simulink model "single_phase_afe"  (R2026b)
settings: Solver=ode23tb  StopTime=param.sim.simlength  FixedStep=param.sim.tc  MaxStep=param.glb_time.tc
values from neighbouring files (symbols this model uses):
  param = struct()    [init_model.m]
undefined symbols (not defined in the file or in its folder): magnitude
libraries: fl_lib x201, nesl_utility x108, igbt_simple_2th_lib x8, single_phase_pwm_modulator x2, dq_vector_pi x2, phase_shift_filter_ccaller x2, pi_ctrl x2, discrete_time_low_pass_filter x2, lithium_ion_battery x1, dclink_for_two_levels x1, three_phase_voltage_with_frt_emulator x1, simulink x1
(part 2 of 7)

== system single_phase_afe/grid/grid_emulator/threephase_vi_measures ==
  Bus Creator : BusCreator  Inputs=6
  Current Sensor : fl_lib/Electrical/Electrical Sensors/Current Sensor
  Current Sensor1 : fl_lib/Electrical/Electrical Sensors/Current Sensor
  Current Sensor2 : fl_lib/Electrical/Electrical Sensors/Current Sensor
  Electrical Reference1 : fl_lib/Electrical/Electrical Elements/Electrical Reference
  Voltage Sensor : fl_lib/Electrical/Electrical Sensors/Voltage Sensor
  Voltage Sensor1 : fl_lib/Electrical/Electrical Sensors/Voltage Sensor
  Voltage Sensor2 : fl_lib/Electrical/Electrical Sensors/Voltage Sensor
  i : Selector  InputPortWidth=6  IndexOptions=Index vector (dialog)  Indices=[4 5 6]  OutputSizes=1  RuntimeRangeChecks=off
  ia_grid : nesl_utility/PS-Simulink Converter  PhysicalDomain=network_engine_domain  SubClassName=ps_output  LeftPortType=input  RightPortType=output  PseudoPeriodic=off  Frequencies=[]  VectorFormat=1-D array  Unit=A  AffineConversion=off
  ib_grid : nesl_utility/PS-Simulink Converter  PhysicalDomain=network_engine_domain  SubClassName=ps_output  LeftPortType=input  RightPortType=output  PseudoPeriodic=off  Frequencies=[]  VectorFormat=1-D array  Unit=A  AffineConversion=off
  ic_grid : nesl_utility/PS-Simulink Converter  PhysicalDomain=network_engine_domain  SubClassName=ps_output  LeftPortType=input  RightPortType=output  PseudoPeriodic=off  Frequencies=[]  VectorFormat=1-D array  Unit=A  AffineConversion=off
  u : Selector  InputPortWidth=6  IndexOptions=Index vector (dialog)  Indices=[1 2 3]  OutputSizes=1  RuntimeRangeChecks=off
  ua_grid : nesl_utility/PS-Simulink Converter  PhysicalDomain=network_engine_domain  SubClassName=ps_output  LeftPortType=input  RightPortType=output  PseudoPeriodic=off  Frequencies=[]  VectorFormat=1-D array  Unit=V  AffineConversion=off
  ub_grid : nesl_utility/PS-Simulink Converter  PhysicalDomain=network_engine_domain  SubClassName=ps_output  LeftPortType=input  RightPortType=output  PseudoPeriodic=off  Frequencies=[]  VectorFormat=1-D array  Unit=V  AffineConversion=off
  uc_grid : nesl_utility/PS-Simulink Converter  PhysicalDomain=network_engine_domain  SubClassName=ps_output  LeftPortType=input  RightPortType=output  PseudoPeriodic=off  Frequencies=[]  VectorFormat=1-D array  Unit=V  AffineConversion=off
  Ua : PMIOPort  Side=Left
  ua : PMIOPort  Port=2  Side=Right
  Ub : PMIOPort  Port=3  Side=Left
  ub : PMIOPort  Port=4  Side=Right
  Uc : PMIOPort  Port=5  Side=Left
  uc : PMIOPort  Port=6  Side=Right
  tag scope: i_abc_line=global, u_abc_line=global
  wires:
  Bus Creator/1 -> i/1, u/1  "vi_data"
  ib_grid/1 -> Bus Creator/5  "ib"
  ia_grid/1 -> Bus Creator/4  "ia"
  ic_grid/1 -> Bus Creator/6  "ic"
  ua_grid/1 -> Bus Creator/1  "ua"
  ub_grid/1 -> Bus Creator/2  "ub"
  uc_grid/1 -> Bus Creator/3  "uc"
  i/1 -> [i_abc_line]
  u/1 -> [u_abc_line]
  connections:
  Current Sensor1/LConn1 -- Ub/RConn1 -- Voltage Sensor1/LConn1
  Electrical Reference1/LConn1 -- Voltage Sensor/RConn2 -- Voltage Sensor2/RConn2 -- Voltage Sensor1/RConn2
  Voltage Sensor/RConn1 -- ua_grid/LConn1
  Current Sensor/RConn2 -- ua/RConn1
  Voltage Sensor1/RConn1 -- ub_grid/LConn1
  Voltage Sensor2/LConn1 -- Current Sensor2/LConn1 -- Uc/RConn1
  Current Sensor/LConn1 -- Ua/RConn1 -- Voltage Sensor/LConn1
  Current Sensor1/RConn2 -- ub/RConn1
  Voltage Sensor2/RConn1 -- uc_grid/LConn1
  ib_grid/LConn1 -- Current Sensor1/RConn1
  ia_grid/LConn1 -- Current Sensor/RConn1
  ic_grid/LConn1 -- Current Sensor2/RConn1
  Current Sensor2/RConn2 -- uc/RConn1

== system single_phase_afe/single_phase_inverter/single phase inverter control/acquisition_and_scaling_current_buffer ==
  in : Inport
  1/Ti5 : Gain  Gain=1/param.afe.buffer.ibez  SaturateOnIntegerOverflow=on  OutDataTypeStr=Inherit: Same as input  ParamDataTypeStr=Inherit: Same as input
  Quantizer : Quantizer  QuantizationInterval=param.meas.adc_quantization
  out : Outport
  wires:
  in/1 -> 1/Ti5/1
  1/Ti5/1 -> Quantizer/1
  Quantizer/1 -> out/1

== system single_phase_afe/single_phase_inverter/single phase inverter control/acquisition_and_scaling_current_with_white_noise ==
  in : Inport
  1/Ti5 : Gain  Gain=1/param.afe.hw.ibez  SaturateOnIntegerOverflow=on  OutDataTypeStr=Inherit: Same as input  ParamDataTypeStr=Inherit: Same as input
  Band-Limited White Noise : simulink/Sources/Band-Limited White Noise  Commented=on  Cov=1e-10  Ts=param.glb_time.tc  seed=[23341]
  Quantizer : Quantizer  QuantizationInterval=param.meas.adc_quantization
  Sum : Sum  Inputs=|++
  current_measure_with-without noise : Scope  NumInputPorts=2
      settings: ActiveDisplayYMinimum=-1.259685411609524  ActiveDisplayYMaximum=1.2603394332468927  DataLoggingVariableName=ScopeData15
  out : Outport
  wires:
  in/1 -> 1/Ti5/1
  1/Ti5/1 -> Sum/1, current_measure_with-without noise/1  "iload_without_noise"
  Sum/1 -> Quantizer/1
  Band-Limited White Noise/1 -> Sum/2
  Quantizer/1 -> out/1, current_measure_with-without noise/2  "iload_with_noise"

== system single_phase_afe/single_phase_inverter/single phase inverter control/acquisition_and_scaling_dc_voltage ==
  in : Inport
  1/Ti3 : Gain  Gain=1/param.afe.hw.udc_nom  SaturateOnIntegerOverflow=on  OutDataTypeStr=Inherit: Same as input  ParamDataTypeStr=Inherit: Same as input
  Quantizer : Quantizer  QuantizationInterval=param.meas.adc_quantization
  out : Outport
  wires:
  in/1 -> 1/Ti3/1
  1/Ti3/1 -> Quantizer/1
  Quantizer/1 -> out/1

== system single_phase_afe/single_phase_inverter/single phase inverter control/acquisition_and_scaling_dc_voltage_buffer ==
  in : Inport
  1/Ti3 : Gain  Gain=1/param.afe.hw.udc_nom  SaturateOnIntegerOverflow=on  OutDataTypeStr=Inherit: Same as input  ParamDataTypeStr=Inherit: Same as input
  Quantizer : Quantizer  QuantizationInterval=param.meas.adc_quantization
  out : Outport
  wires:
  Quantizer/1 -> out/1
  1/Ti3/1 -> Quantizer/1
  in/1 -> 1/Ti3/1

== system single_phase_afe/single_phase_inverter/single phase inverter control/acquisition_and_scaling_grid_voltage_ac ==
  in : Inport
  1/Ti5 : Gain  Gain=1/param.grid.emu.u2bez  SaturateOnIntegerOverflow=on  OutDataTypeStr=Inherit: Same as input  ParamDataTypeStr=Inherit: Same as input
  Quantizer : Quantizer  QuantizationInterval=param.meas.adc_quantization
  out : Outport
  wires:
  Quantizer/1 -> out/1
  1/Ti5/1 -> Quantizer/1
  in/1 -> 1/Ti5/1

== system single_phase_afe/single_phase_inverter/single phase inverter control/acquisition_and_scaling_voltage ==
  in : Inport
  1/Ti5 : Gain  Gain=1/param.afe.hw.ubez  SaturateOnIntegerOverflow=on  OutDataTypeStr=Inherit: Same as input  ParamDataTypeStr=Inherit: Same as input
  Quantizer : Quantizer  QuantizationInterval=param.meas.adc_quantization
  pwm filtering for measure : cstblocks_lti/LTI System  sys=param.afe.ctrl.sogi.flt_beta  IC=[]  PadeOrder=0
  out : Outport
  wires:
  in/1 -> 1/Ti5/1
  pwm filtering for measure/1 -> Quantizer/1
  1/Ti5/1 -> pwm filtering for measure/1
  Quantizer/1 -> out/1

== system single_phase_afe/single_phase_inverter/single phase inverter control/pwm modulator ==
  vout : Inport
  Constant : Constant  Value=0
  Single phase two level PWM generator with global TRGO : single_phase_pwm_modulator/Single phase two level PWM generator with global TRGO  f=param.glb_time.fPWM_AFE  m_up=0.98  m_low=0.02  dead_time=param.glb_time.dead_time_AFE  pos_cmd_gate=18  neg_cmd_gate=-3  polarity=-1  tc=param.glb_time.tc  double_sampling=param.glb_time.TRGO_AFE_double_update
  gate_cmds : Outport
  tag scope: TRGO_AFE_1=global
  wires:
  vout/1 -> Single phase two level PWM generator with global TRGO/3
  Constant/1 -> Single phase two level PWM generator with global TRGO/2
  Single phase two level PWM generator with global TRGO/2 -> gate_cmds/1
  Single phase two level PWM generator with global TRGO/1 -> [TRGO_AFE_1]
  [time_afe_module_1] -> Single phase two level PWM generator with global TRGO/1

== system single_phase_afe/single_phase_inverter/single phase inverter control/pwm modulator_dclink_compensator ==
  vout : Inport
  Constant : Constant  Value=0
  Single phase two level PWM generator with global TRGO : single_phase_pwm_modulator/Single phase two level PWM generator with global TRGO  f=param.glb_time.fPWM_AFE  m_up=0.98  m_low=0.02  dead_time=param.glb_time.dead_time_AFE  pos_cmd_gate=18  neg_cmd_gate=-3  polarity=-1  tc=param.glb_time.tc  double_sampling=param.glb_time.TRGO_AFE_double_update
  gate_cmds : Outport
  wires:
  [time_afe_module_1] -> Single phase two level PWM generator with global TRGO/1
  Single phase two level PWM generator with global TRGO/2 -> gate_cmds/1
  Constant/1 -> Single phase two level PWM generator with global TRGO/2
  vout/1 -> Single phase two level PWM generator with global TRGO/3

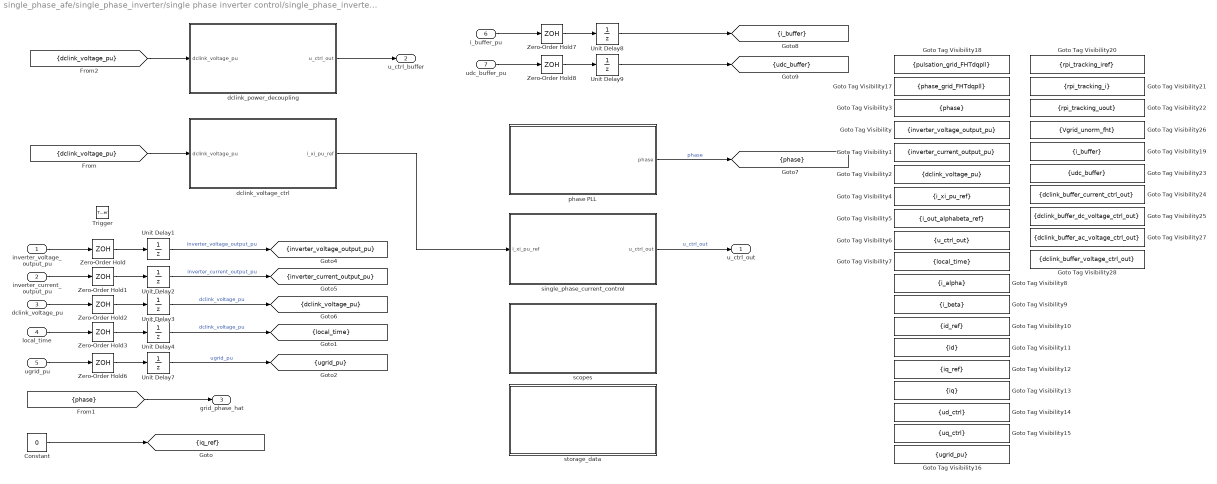
== system single_phase_afe/single_phase_inverter/single phase inverter control/single_phase_inverter_ctrl ==
  inverter_voltage_output_pu : Inport
  inverter_current_output_pu : Inport  Port=2
  dclink_voltage_pu : Inport  Port=3
  local_time : Inport  Port=4
  ugrid_pu : Inport  Port=5
  i_buffer_pu : Inport  Port=6
  udc_buffer_pu : Inport  Port=7
  Trigger : TriggerPort  VariantControl=(inherit)  PortDimensions=1
  Constant : Constant  Value=0
  Goto Tag Visibility : GotoTagVisibility  GotoTag=inverter_voltage_output_pu
  Goto Tag Visibility1 : GotoTagVisibility  GotoTag=inverter_current_output_pu
  Goto Tag Visibility10 : GotoTagVisibility  GotoTag=id_ref
  Goto Tag Visibility11 : GotoTagVisibility  GotoTag=id
  Goto Tag Visibility12 : GotoTagVisibility  GotoTag=iq_ref
  Goto Tag Visibility13 : GotoTagVisibility  GotoTag=iq
  Goto Tag Visibility14 : GotoTagVisibility  GotoTag=ud_ctrl
  Goto Tag Visibility15 : GotoTagVisibility  GotoTag=uq_ctrl
  Goto Tag Visibility16 : GotoTagVisibility  GotoTag=ugrid_pu
  Goto Tag Visibility17 : GotoTagVisibility  GotoTag=phase_grid_FHTdqpll
  Goto Tag Visibility18 : GotoTagVisibility  GotoTag=pulsation_grid_FHTdqpll
  Goto Tag Visibility19 : GotoTagVisibility  GotoTag=i_buffer
  Goto Tag Visibility2 : GotoTagVisibility  GotoTag=dclink_voltage_pu
  Goto Tag Visibility20 : GotoTagVisibility  GotoTag=rpi_tracking_iref
  Goto Tag Visibility21 : GotoTagVisibility  GotoTag=rpi_tracking_i
  Goto Tag Visibility22 : GotoTagVisibility  GotoTag=rpi_tracking_uout
  Goto Tag Visibility23 : GotoTagVisibility  GotoTag=udc_buffer
  Goto Tag Visibility24 : GotoTagVisibility  GotoTag=dclink_buffer_current_ctrl_out
  Goto Tag Visibility25 : GotoTagVisibility  GotoTag=dclink_buffer_dc_voltage_ctrl_out
  Goto Tag Visibility26 : GotoTagVisibility  GotoTag=Vgrid_unorm_fht
  Goto Tag Visibility27 : GotoTagVisibility  GotoTag=dclink_buffer_ac_voltage_ctrl_out
  Goto Tag Visibility28 : GotoTagVisibility  GotoTag=dclink_buffer_voltage_ctrl_out
  Goto Tag Visibility3 : GotoTagVisibility  GotoTag=phase
  Goto Tag Visibility4 : GotoTagVisibility  GotoTag=i_xi_pu_ref
  Goto Tag Visibility5 : GotoTagVisibility  GotoTag=i_out_alphabeta_ref
  Goto Tag Visibility6 : GotoTagVisibility  GotoTag=u_ctrl_out
  Goto Tag Visibility7 : GotoTagVisibility  GotoTag=local_time
  Goto Tag Visibility8 : GotoTagVisibility  GotoTag=i_alpha
  Goto Tag Visibility9 : GotoTagVisibility  GotoTag=i_beta
  Unit Delay{1..4,7..9} (7 alike) : UnitDelay  SampleTime=-1
  Zero-Order Hold{,1..3,6..8} (7 alike) : ZeroOrderHold  SampleTime=-1
  dclink_power_decoupling : Subsystem
  dclink_voltage_ctrl : Subsystem
  phase PLL : Subsystem
  scopes : Subsystem
  single_phase_current_control : Subsystem
  storage_data : Subsystem
  u_ctrl_out : Outport
  u_ctrl_buffer : Outport  Port=2
  grid_phase_hat : Outport  Port=3
  tag scope: dclink_voltage_pu=scoped, i_buffer=scoped, inverter_current_output_pu=scoped, inverter_voltage_output_pu=scoped, iq_ref=scoped, local_time=scoped, phase=scoped, udc_buffer=scoped, ugrid_pu=scoped
  wires:
  inverter_voltage_output_pu/1 -> Zero-Order Hold/1
  inverter_current_output_pu/1 -> Zero-Order Hold1/1
  dclink_voltage_pu/1 -> Zero-Order Hold2/1
  Unit Delay1/1 -> [inverter_voltage_output_pu]  "inverter_voltage_output_pu"
  Unit Delay2/1 -> [inverter_current_output_pu]  "inverter_current_output_pu"
  Unit Delay3/1 -> [dclink_voltage_pu]  "dclink_voltage_pu"
  phase PLL/1(phase) -> [phase]  "phase"
  single_phase_current_control/1(u_ctrl_out) -> u_ctrl_out/1  "u_ctrl_out"
  Zero-Order Hold/1 -> Unit Delay1/1
  Zero-Order Hold1/1 -> Unit Delay2/1
  Zero-Order Hold2/1 -> Unit Delay3/1
  Zero-Order Hold3/1 -> Unit Delay4/1
  Unit Delay4/1 -> [local_time]  "dclink_voltage_pu"
  local_time/1 -> Zero-Order Hold3/1
  ugrid_pu/1 -> Zero-Order Hold6/1
  Zero-Order Hold6/1 -> Unit Delay7/1
  Unit Delay7/1 -> [ugrid_pu]  "ugrid_pu"
  [dclink_voltage_pu] -> dclink_voltage_ctrl/1(dclink_voltage_pu)
  dclink_voltage_ctrl/1(i_xi_pu_ref) -> single_phase_current_control/1(i_xi_pu_ref)
  [phase] -> grid_phase_hat/1
  [dclink_voltage_pu] -> dclink_power_decoupling/1(dclink_voltage_pu)
  dclink_power_decoupling/1(u_ctrl_out) -> u_ctrl_buffer/1
  Zero-Order Hold7/1 -> Unit Delay8/1
  i_buffer_pu/1 -> Zero-Order Hold7/1
  Unit Delay8/1 -> [i_buffer]
  Unit Delay9/1 -> [udc_buffer]
  udc_buffer_pu/1 -> Zero-Order Hold8/1
  Zero-Order Hold8/1 -> Unit Delay9/1
  Constant/1 -> [iq_ref]

== system single_phase_afe/single_phase_inverter/single_phase_inverter/single phase inverter ==
  gate_cmds : Inport
  three_phase_inverter_with_igbt_simple_2th : Subsystem
  uac_out(+) : PMIOPort  Side=Left
  uac_out(-) : PMIOPort  Port=2  Side=Left
  udc(+) : PMIOPort  Port=3  Side=Right
  udc(-) : PMIOPort  Port=4  Side=Right
  wires:
  gate_cmds/1 -> three_phase_inverter_with_igbt_simple_2th/1(gate_cmds)
  connections:
  udc(-)/RConn1 -- three_phase_inverter_with_igbt_simple_2th/LConn2
  udc(+)/RConn1 -- three_phase_inverter_with_igbt_simple_2th/LConn1
  uac_out(+)/RConn1 -- three_phase_inverter_with_igbt_simple_2th/RConn1
  uac_out(-)/RConn1 -- three_phase_inverter_with_igbt_simple_2th/RConn2

== system single_phase_afe/dclink_buffer_ctrl/single_phase_inverter/single phase inverter/three_phase_inverter_with_igbt_simple_2th ==
  gate_cmds : Inport
  full_bridge_with_igbt_simple_2th : Subsystem  mask{vce_sat_m=param.afe.igbt.Vce_sat, v_gamma_m=param.afe.igbt.Vdon_diode, Vth_gate_m=param.afe.igbt.Vth, Vth_gate_hyst_m=0.85, Eon_m=param.afe.igbt.Eon*1000, Eoff_m=param.afe.igbt.Eoff*1000, Err_m=param.afe.igbt.Erec*1000, Ic_ref_m=param.afe.igbt.Ion_sw_losses, Vdc_ref_m=param.afe.igbt.Voff_sw_losses, Vblock_Errf_m=50, rce_on_m=param.afe.igbt.Rce_on*1000, rd_on_m=param.afe.igbt.Rdon_diode*1000, Gce_off_m=1e-6, time_constant_edge_m=param.glb_time.tc, time_constant_ploss_m=1e3, Csnubber_m=param.afe.igbt.Csnubber_zvs, Rsnubber_m=param.afe.igbt.Rsnubber_zvs, rth_switch_JH_m=param.afe.igbt.Rth_switch_JH, rth_switch_HA_m=param.thermal.heatsink.Rth_switch_HA, rth_diode_JH_m=param.afe.igbt.Rth_diode_JH, rth_diode_HA_m=param.thermal.heatsink.Rth_diode_HA, JunctionTermalMass_m=param.afe.igbt.JunctionTermalMass, Tambient_m=param.thermal.Tambient, mass_heatsink_m=param.thermal.heatsink.no_weight, specific_heat_m=param.thermal.heatsink.cp}
      mask prompts: vce_sat_m "Collector-emitter on-stage voltage [V]"; v_gamma_m "Diode forward voltage [V]"; Vth_gate_m "Gate-emitter threshold voltage [V]"; Vth_gate_hyst_m "Half hysteresis band for the switching events [V]"; Eon_m "Turn-on energy at Ic_ref, Vdc_ref [mJ]"; Eoff_m "Turn-off energy at Ic_ref, Vdc_ref [mJ]"; Err_m "Reverse recovery energy at Ic_ref, Vdc_ref [mJ]"; Ic_ref_m "Reference current of the energies [A]"; Vdc_ref_m "Reference voltage of the energies [V]"; Vblock_Errf_m "V block Err"; rce_on_m "IGBT on-state series resistance [mOhm]"; rd_on_m "Diode series resistance [mOhm]"; Gce_off_m "Off-state conductance [1/Ohm]"; time_constant_edge_m "Sample&hold time constant (<< on-time) [us]"; time_constant_ploss_m "Loss averaging time constant (2-5 x Tsw) [us]"; Csnubber_m "Csnubber [F]"; Rsnubber_m "Rsnubber [Ohm]"; rth_switch_JH_m "Thermal impedance Junction-heatsink switch [K/W]"; rth_switch_HA_m "Thermal impedance heatsink-ambient switch[K/W]"; rth_diode_JH_m "Thermal impedance Junction-heatsink diode [K/W]"; rth_diode_HA_m "Thermal impedance heatsink-ambient diode [K/W]"; JunctionTermalMass_m "Junction Thermal Mass [J/K]"; Tambient_m "Ambient temperature [degC]"; mass_heatsink_m "Mass heatsink [kg]"; specific_heat_m "Specific heat capacity of the heatsink [J/K/Kg]"
  u1 : PMIOPort  Side=Right
  u2 : PMIOPort  Port=2  Side=Right
  udc(+) : PMIOPort  Port=3  Side=Left
  udc(-) : PMIOPort  Port=4  Side=Left
  wires:
  gate_cmds/1 -> full_bridge_with_igbt_simple_2th/1(gate_cmds)
  connections:
  u1/RConn1 -- full_bridge_with_igbt_simple_2th/RConn1
  u2/RConn1 -- full_bridge_with_igbt_simple_2th/RConn2
  udc(-)/RConn1 -- full_bridge_with_igbt_simple_2th/LConn2
  udc(+)/RConn1 -- full_bridge_with_igbt_simple_2th/LConn1

== system single_phase_afe/single_phase_inverter/single phase inverter control/single_phase_inverter_ctrl/dclink_power_decoupling ==
  dclink_voltage_pu : Inport
  dclink_decoupling_ctrl : Subsystem
  idc_buffer_ctrl : Subsystem
  udc_buffer_ctrl : Subsystem
  u_ctrl_out : Outport
  wires:
  idc_buffer_ctrl/1(u_ctrl_out) -> u_ctrl_out/1, dclink_decoupling_ctrl/3(u_ctrl_out)  "u_ctrl_out"
  [udc_buffer] -> udc_buffer_ctrl/1(udc_buffer_pu)
  udc_buffer_ctrl/1(i_dc_buffer_ref) -> dclink_decoupling_ctrl/1(i_dc_buffer_ref)  "i_dc_buffer_ref"
  dclink_voltage_pu/1 -> dclink_decoupling_ctrl/2(udc_dclink_pu)  "udc_dclink_pu"
  dclink_decoupling_ctrl/1(i_buffer_ref) -> idc_buffer_ctrl/1(i_buffer_ref)  "i_buffer_ref"

== system single_phase_afe/single_phase_inverter/single phase inverter control/single_phase_inverter_ctrl/dclink_voltage_ctrl ==
  dclink_voltage_pu : Inport
  1/Ti : Gain  Gain=param.afe.ctrl.kp_udc  SaturateOnIntegerOverflow=on  OutDataTypeStr=Inherit: Same as input  ParamDataTypeStr=Inherit: Same as input
  Gain : Gain  Gain=-1
  Saturation : Saturate  UpperLimit=param.afe.ctrl.i_ref_lim  LowerLimit=-param.afe.ctrl.i_ref_lim
  Sum1 : Sum  Inputs=+++  SaturateOnIntegerOverflow=on
  Sum2 : Sum  Inputs=-+  SaturateOnIntegerOverflow=on
  Sum3 : Sum  Inputs=-+  SaturateOnIntegerOverflow=on
  To Workspace1 : ToWorkspace  VariableName=udc_pu_sim_mod1  SampleTime=-1
      settings: MaxDataPoints=param.glb_time.Ns_afe
  To Workspace3 : ToWorkspace  VariableName=udc_pu_ref_sim_mod1  SampleTime=-1
      settings: MaxDataPoints=param.glb_time.Ns_afe
  Unit Delay4 : UnitDelay  SampleTime=-1
  discrete-time-low-pass-filter1 : discrete_time_low_pass_filter/discrete-time-low-pass-filter  tau=param.afe.ctrl.tau_udc_ref  ts=param.glb_time.ts_afe
  kp : Gain  Gain=param.afe.ctrl.ki_udc*param.glb_time.ts_afe  SaturateOnIntegerOverflow=on  OutDataTypeStr=Inherit: Same as input  ParamDataTypeStr=Inherit: Same as input
  udc_norm_ref : Step  Time=param.afe.ctrl.t_udc_ref  FinalValue=param.afe.ctrl.udc_pu_ref
  udc_tracking : Scope  NumInputPorts=3
      settings: ActiveDisplayYMinimum=-2.0073730468749997  ActiveDisplayYMaximum=1.5663574218749998  DataLoggingVariableName=ScopeData8
  i_xi_pu_ref : Outport
  wires:
  1/Ti/1 -> Sum1/1, Sum3/1
  kp/1 -> Sum1/2
  Sum3/1 -> Unit Delay4/1
  Unit Delay4/1 -> Sum1/3
  udc_norm_ref/1 -> discrete-time-low-pass-filter1/1
  dclink_voltage_pu/1 -> Sum2/1, To Workspace1/1, udc_tracking/2  "udc_pu"
  Sum2/1 -> kp/1, 1/Ti/1
  Sum1/1 -> Saturation/1
  Saturation/1 -> Sum3/2, Gain/1
  Gain/1 -> udc_tracking/3, i_xi_pu_ref/1  "i_xi_pu_ref"
  discrete-time-low-pass-filter1/1 -> To Workspace3/1, udc_tracking/1, Sum2/2  "udc_pu_ref"

== system single_phase_afe/single_phase_inverter/single phase inverter control/single_phase_inverter_ctrl/phase PLL ==
  FHT-PLL : Subsystem
  FHTdqpll : Scope  NumInputPorts=2
      settings: ActiveDisplayYMinimum=-1.624956414103508  ActiveDisplayYMaximum=4.624995157122612  DataLoggingVariableName=ScopeData3
  phase : Outport
  tag scope: phase_grid_FHTdqpll=scoped, pulsation_grid_FHTdqpll=scoped
  wires:
  FHT-PLL/1(phase_grid_fht_pll) -> [phase_grid_FHTdqpll]
  FHT-PLL/2(omega_grid_fht_pll) -> [pulsation_grid_FHTdqpll]
  [ugrid_pu] -> FHT-PLL/1(ug_abc_pu)
  [phase_grid_FHTdqpll] -> FHTdqpll/1  "phase_grid_FHTdqpll"
  [pulsation_grid_FHTdqpll] -> FHTdqpll/2  "pulsation_grid_FHTdqpll"
  [phase_grid_FHTdqpll] -> phase/1

== system single_phase_afe/single_phase_inverter/single phase inverter control/single_phase_inverter_ctrl/scopes ==
  Bus Creator1 : BusCreator  Inputs=3
  Bus Creator2 : BusCreator  Inputs=2
  Bus Creator3 : BusCreator  Inputs=2
  Bus Creator4 : BusCreator  Inputs=2
  single phase inverter tracking current scope 1 : Scope  NumInputPorts=2
      settings: ActiveDisplayYMinimum=-2.05401611328125  ActiveDisplayYMaximum=4.66778564453125  DataLoggingVariableName=ScopeData12
  single phase inverter tracking current scope 2 : Scope  NumInputPorts=2
      settings: ActiveDisplayYMinimum=-1.2603759765625  ActiveDisplayYMaximum=1.2652587890625  DataLoggingVariableName=ScopeData2
  wires:
  Bus Creator1/1 -> single phase inverter tracking current scope 1/2  "is_tracking"
  [i_out_alphabeta_ref] -> Bus Creator1/2  "i_out_inverter_pu_ref"
  [inverter_current_output_pu] -> Bus Creator1/3  "inverter_current_output_pu"
  [inverter_voltage_output_pu] -> Bus Creator2/1  "inverter_voltage_output_pu"
  Bus Creator2/1 -> single phase inverter tracking current scope 1/1  "load"
  [i_xi_pu_ref] -> Bus Creator1/1  "inverter_current_output_pu_reference"
  [inverter_current_output_pu] -> Bus Creator2/2  "inverter_current_output_pu"
  [u_ctrl_out] -> Bus Creator3/1  "u_ctrl_out"
  [inverter_voltage_output_pu] -> Bus Creator3/2  "inverter_voltage_output_pu"
  Bus Creator3/1 -> single phase inverter tracking current scope 2/2  "u_load"
  [inverter_current_output_pu] -> Bus Creator4/2  "inverter_current_output_pu"
  [i_out_alphabeta_ref] -> Bus Creator4/1  "i_out_alphabeta_ref"
  Bus Creator4/1 -> single phase inverter tracking current scope 2/1  "i_load"

== system single_phase_afe/single_phase_inverter/single phase inverter control/single_phase_inverter_ctrl/single_phase_current_control ==
  i_xi_pu_ref : Inport
  current_reference_generation : Subsystem
  dqpi_current_controller : Subsystem
  u_ctrl_out : Outport
  tag scope: i_out_alphabeta_ref=scoped, i_xi_pu_ref=scoped, u_ctrl_out=scoped
  wires:
  current_reference_generation/1(is_ref) -> [i_out_alphabeta_ref]  "i_out_inverter_pu_ref"
  dqpi_current_controller/1(u_out) -> u_ctrl_out/1, [u_ctrl_out]  "u_ctrl_out"
  [phase] -> current_reference_generation/2(phase)
  i_xi_pu_ref/1 -> current_reference_generation/1(i_xi_pu_ref), [i_xi_pu_ref]
  current_reference_generation/2(id_ref) -> dqpi_current_controller/1(id_ref)

== system single_phase_afe/single_phase_inverter/single phase inverter control/single_phase_inverter_ctrl/storage_data ==
  To Workspace : ToWorkspace  VariableName=inverter_voltage_output_pu_sim  SampleTime=-1
      settings: MaxDataPoints=param.glb_time.Ns_afe  Save2DSignal=2-D array (concatenate along first dimension)
  To Workspace1 : ToWorkspace  VariableName=inverter_current_output_pu_sim  SampleTime=-1
      settings: MaxDataPoints=param.glb_time.Ns_afe  Save2DSignal=2-D array (concatenate along first dimension)
  To Workspace10 : ToWorkspace  VariableName=dclink_buffer_ac_voltage_ctrl_out_sim  SampleTime=-1
      settings: MaxDataPoints=param.glb_time.Ns_afe  Save2DSignal=2-D array (concatenate along first dimension)
  To Workspace11 : ToWorkspace  VariableName=iq_pu_sim  SampleTime=-1
      settings: MaxDataPoints=param.glb_time.Ns_afe  Save2DSignal=2-D array (concatenate along first dimension)
  To Workspace12 : ToWorkspace  VariableName=ud_ctrl_out_sim  SampleTime=-1
      settings: MaxDataPoints=param.glb_time.Ns_afe  Save2DSignal=2-D array (concatenate along first dimension)
  To Workspace13 : ToWorkspace  VariableName=uq_ctrl_out_sim  SampleTime=-1
      settings: MaxDataPoints=param.glb_time.Ns_afe  Save2DSignal=2-D array (concatenate along first dimension)
  To Workspace14 : ToWorkspace  VariableName=dclink_buffer_voltage_ctrl_out_sim  SampleTime=-1
      settings: MaxDataPoints=param.glb_time.Ns_afe  Save2DSignal=2-D array (concatenate along first dimension)
  To Workspace19 : ToWorkspace  VariableName=dclink_buffer_current_ctrl_out_sim  SampleTime=-1
      settings: MaxDataPoints=param.glb_time.Ns_afe  Save2DSignal=2-D array (concatenate along first dimension)
  To Workspace2 : ToWorkspace  VariableName=inverter_current_output_pu_reference_sim  SampleTime=-1
      settings: MaxDataPoints=param.glb_time.Ns_afe  Save2DSignal=2-D array (concatenate along first dimension)
  To Workspace20 : ToWorkspace  VariableName=dclink_buffer_dc_voltage_ctrl_out_sim  SampleTime=-1
      settings: MaxDataPoints=param.glb_time.Ns_afe  Save2DSignal=2-D array (concatenate along first dimension)
  To Workspace3 : ToWorkspace  VariableName=i_out_inverter_pu_ref_sim  SampleTime=-1
      settings: MaxDataPoints=param.glb_time.Ns_afe  Save2DSignal=2-D array (concatenate along first dimension)
  To Workspace4 : ToWorkspace  VariableName=u_ctrl_out_sim  SampleTime=-1
      settings: MaxDataPoints=param.glb_time.Ns_afe  Save2DSignal=2-D array (concatenate along first dimension)
  To Workspace5 : ToWorkspace  VariableName=time_ts_inv_sim  SampleTime=-1
      settings: MaxDataPoints=param.glb_time.Ns_afe  Save2DSignal=2-D array (concatenate along first dimension)
  To Workspace6 : ToWorkspace  VariableName=i_alpha_pu_sim  SampleTime=-1
      settings: MaxDataPoints=param.glb_time.Ns_afe  Save2DSignal=2-D array (concatenate along first dimension)
  To Workspace7 : ToWorkspace  VariableName=i_beta_pu_sim  SampleTime=-1
      settings: MaxDataPoints=param.glb_time.Ns_afe  Save2DSignal=2-D array (concatenate along first dimension)
  To Workspace8 : ToWorkspace  VariableName=id_pu_ref_sim  SampleTime=-1
      settings: MaxDataPoints=param.glb_time.Ns_afe  Save2DSignal=2-D array (concatenate along first dimension)
  To Workspace9 : ToWorkspace  VariableName=id_pu_sim  SampleTime=-1
      settings: MaxDataPoints=param.glb_time.Ns_afe  Save2DSignal=2-D array (concatenate along first dimension)
  wires:
  [inverter_voltage_output_pu] -> To Workspace/1  "inverter_voltage_output_pu"
  [inverter_current_output_pu] -> To Workspace1/1  "inverter_current_output_pu"
  [i_xi_pu_ref] -> To Workspace2/1  "inverter_current_output_pu_reference"
  [i_out_alphabeta_ref] -> To Workspace3/1  "i_out_inverter_pu_ref"
  [u_ctrl_out] -> To Workspace4/1  "u_ctrl_out"
  [local_time] -> To Workspace5/1
  [i_alpha] -> To Workspace6/1
  [i_beta] -> To Workspace7/1
  [id_ref] -> To Workspace8/1
  [id] -> To Workspace9/1
  [iq] -> To Workspace11/1
  [ud_ctrl] -> To Workspace12/1
  [uq_ctrl] -> To Workspace13/1
  [dclink_buffer_current_ctrl_out] -> To Workspace19/1
  [dclink_buffer_dc_voltage_ctrl_out] -> To Workspace20/1
  [dclink_buffer_ac_voltage_ctrl_out] -> To Workspace10/1
  [dclink_buffer_voltage_ctrl_out] -> To Workspace14/1

== system single_phase_afe/single_phase_inverter/single_phase_inverter/single phase inverter/three_phase_inverter_with_igbt_simple_2th ==
  gate_cmds : Inport
  Bus Selector : BusSelector  OutputSignals=module_1.igbt_ploss_Q2,module_1.igbt_voltage_Q2,module_1.igbt_current_Q2,module_1.igbt_JH_temp_Q2,module_1.igbt_HA_temp_Q2
  Bus Selector1 : BusSelector  OutputSignals=module_1.igbt_ploss_Q1,module_1.igbt_voltage_Q1,module_1.igbt_current_Q1,module_1.igbt_JH_temp_Q1,module_1.igbt_HA_temp_Q1
  Bus Selector2 : BusSelector  OutputSignals=module_2.igbt_ploss_Q3,module_2.igbt_voltage_Q3,module_2.igbt_current_Q3,module_2.igbt_JH_temp_Q3,module_2.igbt_HA_temp_Q3
  Bus Selector3 : BusSelector  OutputSignals=module_1.diode_ploss_Q1,module_1.diode_JH_temp_Q1,module_1.diode_HA_temp_Q1,module_1.diode_current_Q1
  full_bridge_with_igbt_simple_2th : Subsystem  mask{vce_sat_m=param.afe.igbt.Vce_sat, v_gamma_m=param.afe.igbt.Vdon_diode, Vth_gate_m=param.afe.igbt.Vth, Vth_gate_hyst_m=0.85, Eon_m=param.afe.igbt.Eon*1000, Eoff_m=param.afe.igbt.Eoff*1000, Err_m=param.afe.igbt.Erec*1000, Ic_ref_m=param.afe.igbt.Ion_sw_losses, Vdc_ref_m=param.afe.igbt.Voff_sw_losses, Vblock_Errf_m=50, rce_on_m=param.afe.igbt.Rce_on*1000, rd_on_m=param.afe.igbt.Rdon_diode*1000, Gce_off_m=1e-6, time_constant_edge_m=param.glb_time.tc, time_constant_ploss_m=1e3, Csnubber_m=param.afe.igbt.Csnubber_zvs, Rsnubber_m=param.afe.igbt.Rsnubber_zvs, rth_switch_JH_m=param.afe.igbt.Rth_switch_JH, rth_switch_HA_m=param.thermal.heatsink.Rth_switch_HA, rth_diode_JH_m=param.afe.igbt.Rth_diode_JH, rth_diode_HA_m=param.thermal.heatsink.Rth_diode_HA, JunctionTermalMass_m=param.afe.igbt.JunctionTermalMass, Tambient_m=param.thermal.Tambient, mass_heatsink_m=param.thermal.heatsink.no_weight, specific_heat_m=param.thermal.heatsink.cp}
      mask prompts: vce_sat_m "Collector-emitter on-stage voltage [V]"; v_gamma_m "Diode forward voltage [V]"; Vth_gate_m "Gate-emitter threshold voltage [V]"; Vth_gate_hyst_m "Half hysteresis band for the switching events [V]"; Eon_m "Turn-on energy at Ic_ref, Vdc_ref [mJ]"; Eoff_m "Turn-off energy at Ic_ref, Vdc_ref [mJ]"; Err_m "Reverse recovery energy at Ic_ref, Vdc_ref [mJ]"; Ic_ref_m "Reference current of the energies [A]"; Vdc_ref_m "Reference voltage of the energies [V]"; Vblock_Errf_m "V block Err"; rce_on_m "IGBT on-state series resistance [mOhm]"; rd_on_m "Diode series resistance [mOhm]"; Gce_off_m "Off-state conductance [1/Ohm]"; time_constant_edge_m "Sample&hold time constant (<< on-time) [us]"; time_constant_ploss_m "Loss averaging time constant (2-5 x Tsw) [us]"; Csnubber_m "Csnubber [F]"; Rsnubber_m "Rsnubber [Ohm]"; rth_switch_JH_m "Thermal impedance Junction-heatsink switch [K/W]"; rth_switch_HA_m "Thermal impedance heatsink-ambient switch[K/W]"; rth_diode_JH_m "Thermal impedance Junction-heatsink diode [K/W]"; rth_diode_HA_m "Thermal impedance heatsink-ambient diode [K/W]"; JunctionTermalMass_m "Junction Thermal Mass [J/K]"; Tambient_m "Ambient temperature [degC]"; mass_heatsink_m "Mass heatsink [kg]"; specific_heat_m "Specific heat capacity of the heatsink [J/K/Kg]"
  u1 : PMIOPort  Side=Right
  u2 : PMIOPort  Port=2  Side=Right
  udc(+) : PMIOPort  Port=3  Side=Left
  udc(-) : PMIOPort  Port=4  Side=Left
  tag scope: diode_HA_temp_afeQ1=global, diode_JH_temp_afeQ1=global, diode_current_afeQ1=global, diode_ploss_afeQ1=global, igbt_HA_temp_afeQ1=global, igbt_HA_temp_afeQ2=global, igbt_HA_temp_afeQ3=global, igbt_JH_temp_afeQ1=global, igbt_JH_temp_afeQ2=global, igbt_JH_temp_afeQ3=global, igbt_current_afeQ1=global, igbt_current_afeQ2=global, igbt_current_afeQ3=global, igbt_ploss_afeQ1=global, igbt_ploss_afeQ2=global, igbt_ploss_afeQ3=global, igbt_voltage_afeQ1=global, igbt_voltage_afeQ2=global, igbt_voltage_afeQ3=global
  wires:
  gate_cmds/1 -> full_bridge_with_igbt_simple_2th/1(gate_cmds)
  Bus Selector3/3 -> [diode_HA_temp_afeQ1]  "<diode_HA_temp_Q1>"
  Bus Selector/1 -> [igbt_ploss_afeQ2]  "<igbt_ploss_Q2>"
  Bus Selector3/2 -> [diode_JH_temp_afeQ1]  "<diode_JH_temp_Q1>"
  Bus Selector1/2 -> [igbt_voltage_afeQ1]  "<igbt_voltage_Q1>"
  Bus Selector/2 -> [igbt_voltage_afeQ2]  "<igbt_voltage_Q2>"
  Bus Selector/5 -> [igbt_HA_temp_afeQ2]  "<igbt_HA_temp_Q2>"
  Bus Selector2/5 -> [igbt_HA_temp_afeQ3]  "<igbt_HA_temp_Q3>"
  Bus Selector2/2 -> [igbt_voltage_afeQ3]  "<igbt_voltage_Q3>"
  Bus Selector/4 -> [igbt_JH_temp_afeQ2]  "<igbt_JH_temp_Q2>"
  Bus Selector1/4 -> [igbt_JH_temp_afeQ1]  "<igbt_JH_temp_Q1>"
  Bus Selector3/1 -> [diode_ploss_afeQ1]  "<diode_ploss_Q1>"
  Bus Selector2/4 -> [igbt_JH_temp_afeQ3]  "<igbt_JH_temp_Q3>"
  Bus Selector2/3 -> [igbt_current_afeQ3]  "<igbt_current_Q3>"
  full_bridge_with_igbt_simple_2th/1(m) -> Bus Selector2/1, Bus Selector/1, Bus Selector3/1, Bus Selector1/1
  Bus Selector1/3 -> [igbt_current_afeQ1]  "<igbt_current_Q1>"
  Bus Selector/3 -> [igbt_current_afeQ2]  "<igbt_current_Q2>"
  Bus Selector1/5 -> [igbt_HA_temp_afeQ1]  "<igbt_HA_temp_Q1>"
  Bus Selector2/1 -> [igbt_ploss_afeQ3]  "<igbt_ploss_Q3>"
  Bus Selector1/1 -> [igbt_ploss_afeQ1]  "<igbt_ploss_Q1>"
  Bus Selector3/4 -> [diode_current_afeQ1]  "<diode_current_Q1>"
  connections:
  u1/RConn1 -- full_bridge_with_igbt_simple_2th/RConn1
  u2/RConn1 -- full_bridge_with_igbt_simple_2th/RConn2
  udc(-)/RConn1 -- full_bridge_with_igbt_simple_2th/LConn2
  udc(+)/RConn1 -- full_bridge_with_igbt_simple_2th/LConn1

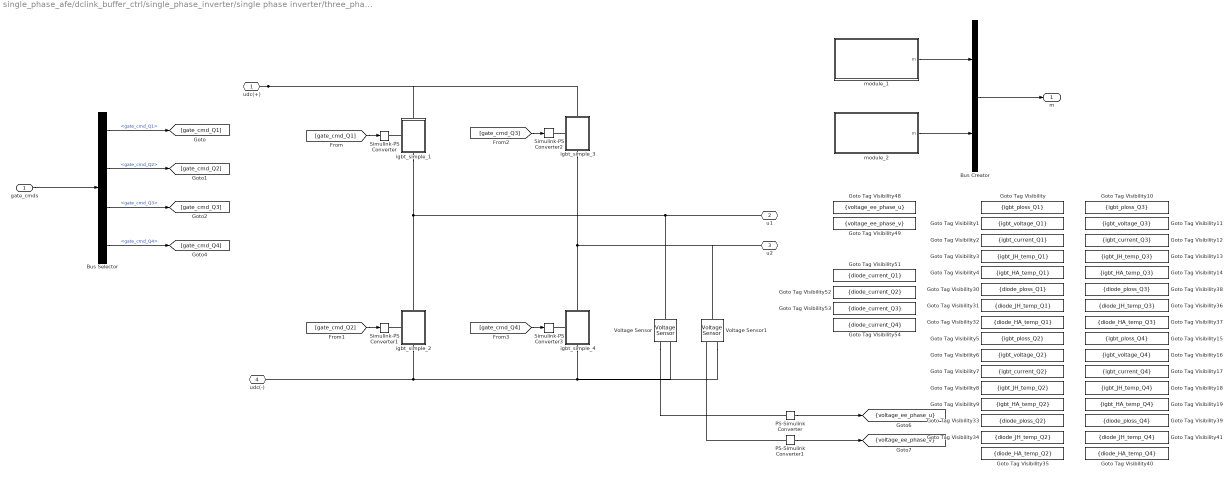
== system single_phase_afe/dclink_buffer_ctrl/single_phase_inverter/single phase inverter/three_phase_inverter_with_igbt_simple_2th/full_bridge_with_igbt_simple_2th ==
  gate_cmds : Inport
  Bus Creator : BusCreator  Inputs=2
  Bus Selector : BusSelector  OutputSignals=gate_cmd_Q1,gate_cmd_Q2,gate_cmd_Q3,gate_cmd_Q4
  Goto Tag Visibility : GotoTagVisibility  GotoTag=igbt_ploss_Q1
  Goto Tag Visibility1 : GotoTagVisibility  GotoTag=igbt_voltage_Q1
  Goto Tag Visibility10 : GotoTagVisibility  GotoTag=igbt_ploss_Q3
  Goto Tag Visibility11 : GotoTagVisibility  GotoTag=igbt_voltage_Q3
  Goto Tag Visibility12 : GotoTagVisibility  GotoTag=igbt_current_Q3
  Goto Tag Visibility13 : GotoTagVisibility  GotoTag=igbt_JH_temp_Q3
  Goto Tag Visibility14 : GotoTagVisibility  GotoTag=igbt_HA_temp_Q3
  Goto Tag Visibility15 : GotoTagVisibility  GotoTag=igbt_ploss_Q4
  Goto Tag Visibility16 : GotoTagVisibility  GotoTag=igbt_voltage_Q4
  Goto Tag Visibility17 : GotoTagVisibility  GotoTag=igbt_current_Q4
  Goto Tag Visibility18 : GotoTagVisibility  GotoTag=igbt_JH_temp_Q4
  Goto Tag Visibility19 : GotoTagVisibility  GotoTag=igbt_HA_temp_Q4
  Goto Tag Visibility2 : GotoTagVisibility  GotoTag=igbt_current_Q1
  Goto Tag Visibility3 : GotoTagVisibility  GotoTag=igbt_JH_temp_Q1
  Goto Tag Visibility30 : GotoTagVisibility  GotoTag=diode_ploss_Q1
  Goto Tag Visibility31 : GotoTagVisibility  GotoTag=diode_JH_temp_Q1
  Goto Tag Visibility32 : GotoTagVisibility  GotoTag=diode_HA_temp_Q1
  Goto Tag Visibility33 : GotoTagVisibility  GotoTag=diode_ploss_Q2
  Goto Tag Visibility34 : GotoTagVisibility  GotoTag=diode_JH_temp_Q2
  Goto Tag Visibility35 : GotoTagVisibility  GotoTag=diode_HA_temp_Q2
  Goto Tag Visibility36 : GotoTagVisibility  GotoTag=diode_JH_temp_Q3
  Goto Tag Visibility37 : GotoTagVisibility  GotoTag=diode_HA_temp_Q3
  Goto Tag Visibility38 : GotoTagVisibility  GotoTag=diode_ploss_Q3
  Goto Tag Visibility39 : GotoTagVisibility  GotoTag=diode_ploss_Q4
  Goto Tag Visibility4 : GotoTagVisibility  GotoTag=igbt_HA_temp_Q1
  Goto Tag Visibility40 : GotoTagVisibility  GotoTag=diode_HA_temp_Q4
  Goto Tag Visibility41 : GotoTagVisibility  GotoTag=diode_JH_temp_Q4
  Goto Tag Visibility48 : GotoTagVisibility  GotoTag=voltage_ee_phase_u
  Goto Tag Visibility49 : GotoTagVisibility  GotoTag=voltage_ee_phase_v
  Goto Tag Visibility5 : GotoTagVisibility  GotoTag=igbt_ploss_Q2
  Goto Tag Visibility51 : GotoTagVisibility  GotoTag=diode_current_Q1
  Goto Tag Visibility52 : GotoTagVisibility  GotoTag=diode_current_Q2
  Goto Tag Visibility53 : GotoTagVisibility  GotoTag=diode_current_Q3
  Goto Tag Visibility54 : GotoTagVisibility  GotoTag=diode_current_Q4
  Goto Tag Visibility6 : GotoTagVisibility  GotoTag=igbt_voltage_Q2
  Goto Tag Visibility7 : GotoTagVisibility  GotoTag=igbt_current_Q2
  Goto Tag Visibility8 : GotoTagVisibility  GotoTag=igbt_JH_temp_Q2
  Goto Tag Visibility9 : GotoTagVisibility  GotoTag=igbt_HA_temp_Q2
  PS-Simulink Converter : nesl_utility/PS-Simulink Converter  PhysicalDomain=network_engine_domain  SubClassName=ps_output  LeftPortType=input  RightPortType=output  PseudoPeriodic=off  Frequencies=[]  VectorFormat=1-D array  Unit=V  AffineConversion=off
  PS-Simulink Converter1 : nesl_utility/PS-Simulink Converter  PhysicalDomain=network_engine_domain  SubClassName=ps_output  LeftPortType=input  RightPortType=output  PseudoPeriodic=off  Frequencies=[]  VectorFormat=1-D array  Unit=V  AffineConversion=off
  Simulink-PS Converter{,1..3} (4 alike) : nesl_utility/Simulink-PS Converter  PhysicalDomain=network_engine_domain  SubClassName=ps_input  LeftPortType=input  RightPortType=output  PseudoPeriodic=off  Frequencies=[]  NoiseDistribution=none  NoiseParameters=[]  Unit=V  AffineConversion=off  FilteringAndDerivatives=provide  SimscapeFilterOrder=1  InputFilterTimeConstant=0.001  UdotUserProvided=0
  Voltage Sensor : fl_lib/Electrical/Electrical Sensors/Voltage Sensor
  Voltage Sensor1 : fl_lib/Electrical/Electrical Sensors/Voltage Sensor
  igbt_simple_1 : Subsystem
      settings: PortSchema="{\"entries\":[{\"content\":{\"sides\":[{\"content\":{\"connectorIds\":[\"LConn1\"]},\"type\":\"ConnectorPlacement.EquallySpacedRectSide\",\"uuid\":\"9277da8d-d460-43e6-8478-dd662f15d226\"},{\"content\":{\"connectorIds\":[],\"side\":\"RIGHT\"},\"type\":\"ConnectorPlacement.EquallySpacedRectSide\",\"uuid\":\"a7ece396-f1d9-4f4f-a05b-db1fc65d6e1d\"},{\"content\":{\"connectorIds\":[\"LConn2\"],\"side\":\"TOP\"},\"type\":\"ConnectorPlacement.EquallySpacedRectSide\",\"uuid\":\"fdd70777-e9cf-4317-afb6-cae87f75d5b0\"},{\"content\":{\"connectorIds\":[\"RConn1\"],\"side\":\"BOTTOM\"},\"type\":\"ConnectorPlacement.EquallySpacedRectSide\",\"uuid\":\"2353ed68-b1a1-4775-9ca9-31e268d5443b\"}]},\"type\":\"ConnectorPlacement.EquallySpacedConnector\",\"uuid\":\"d5479f4c-4e65-4791-adcb-73df11f88590\"}],\"packageUris\":[\"http://schema.mathworks.com/mf0/Connector/R2020b\"],\"version\":\"1.0\"}"
  igbt_simple_2 : Subsystem
      settings: PortSchema="{\"entries\":[{\"content\":{\"sides\":[{\"content\":{\"connectorIds\":[\"LConn1\"]},\"type\":\"ConnectorPlacement.EquallySpacedRectSide\",\"uuid\":\"9277da8d-d460-43e6-8478-dd662f15d226\"},{\"content\":{\"connectorIds\":[],\"side\":\"RIGHT\"},\"type\":\"ConnectorPlacement.EquallySpacedRectSide\",\"uuid\":\"a7ece396-f1d9-4f4f-a05b-db1fc65d6e1d\"},{\"content\":{\"connectorIds\":[\"LConn2\"],\"side\":\"TOP\"},\"type\":\"ConnectorPlacement.EquallySpacedRectSide\",\"uuid\":\"fdd70777-e9cf-4317-afb6-cae87f75d5b0\"},{\"content\":{\"connectorIds\":[\"RConn1\"],\"side\":\"BOTTOM\"},\"type\":\"ConnectorPlacement.EquallySpacedRectSide\",\"uuid\":\"2353ed68-b1a1-4775-9ca9-31e268d5443b\"}]},\"type\":\"ConnectorPlacement.EquallySpacedConnector\",\"uuid\":\"d5479f4c-4e65-4791-adcb-73df11f88590\"}],\"packageUris\":[\"http://schema.mathworks.com/mf0/Connector/R2020b\"],\"version\":\"1.0\"}"
  igbt_simple_3 : Subsystem
      settings: PortSchema="{\"entries\":[{\"content\":{\"sides\":[{\"content\":{\"connectorIds\":[\"LConn1\"]},\"type\":\"ConnectorPlacement.EquallySpacedRectSide\",\"uuid\":\"9277da8d-d460-43e6-8478-dd662f15d226\"},{\"content\":{\"connectorIds\":[],\"side\":\"RIGHT\"},\"type\":\"ConnectorPlacement.EquallySpacedRectSide\",\"uuid\":\"a7ece396-f1d9-4f4f-a05b-db1fc65d6e1d\"},{\"content\":{\"connectorIds\":[\"LConn2\"],\"side\":\"TOP\"},\"type\":\"ConnectorPlacement.EquallySpacedRectSide\",\"uuid\":\"fdd70777-e9cf-4317-afb6-cae87f75d5b0\"},{\"content\":{\"connectorIds\":[\"RConn1\"],\"side\":\"BOTTOM\"},\"type\":\"ConnectorPlacement.EquallySpacedRectSide\",\"uuid\":\"2353ed68-b1a1-4775-9ca9-31e268d5443b\"}]},\"type\":\"ConnectorPlacement.EquallySpacedConnector\",\"uuid\":\"d5479f4c-4e65-4791-adcb-73df11f88590\"}],\"packageUris\":[\"http://schema.mathworks.com/mf0/Connector/R2020b\"],\"version\":\"1.0\"}"
  igbt_simple_4 : Subsystem
      settings: PortSchema="{\"entries\":[{\"content\":{\"sides\":[{\"content\":{\"connectorIds\":[\"LConn1\"]},\"type\":\"ConnectorPlacement.EquallySpacedRectSide\",\"uuid\":\"9277da8d-d460-43e6-8478-dd662f15d226\"},{\"content\":{\"connectorIds\":[],\"side\":\"RIGHT\"},\"type\":\"ConnectorPlacement.EquallySpacedRectSide\",\"uuid\":\"a7ece396-f1d9-4f4f-a05b-db1fc65d6e1d\"},{\"content\":{\"connectorIds\":[\"LConn2\"],\"side\":\"TOP\"},\"type\":\"ConnectorPlacement.EquallySpacedRectSide\",\"uuid\":\"fdd70777-e9cf-4317-afb6-cae87f75d5b0\"},{\"content\":{\"connectorIds\":[\"RConn1\"],\"side\":\"BOTTOM\"},\"type\":\"ConnectorPlacement.EquallySpacedRectSide\",\"uuid\":\"2353ed68-b1a1-4775-9ca9-31e268d5443b\"}]},\"type\":\"ConnectorPlacement.EquallySpacedConnector\",\"uuid\":\"d5479f4c-4e65-4791-adcb-73df11f88590\"}],\"packageUris\":[\"http://schema.mathworks.com/mf0/Connector/R2020b\"],\"version\":\"1.0\"}"
  module_1 : Subsystem
  module_2 : Subsystem
  udc(+) : PMIOPort  Side=Left
  u1 : PMIOPort  Port=2  Side=Right
  u2 : PMIOPort  Port=3  Side=Right
  udc(-) : PMIOPort  Port=4  Side=Left
  m : Outport
  tag scope: voltage_ee_phase_u=scoped, voltage_ee_phase_v=scoped
  wires:
  module_1/1(m) -> Bus Creator/1
  Bus Creator/1 -> m/1
  module_2/1(m) -> Bus Creator/2
  PS-Simulink Converter1/1 -> [voltage_ee_phase_v]
  PS-Simulink Converter/1 -> [voltage_ee_phase_u]
  [gate_cmd_Q3] -> Simulink-PS Converter2/1
  [gate_cmd_Q4] -> Simulink-PS Converter3/1
  [gate_cmd_Q2] -> Simulink-PS Converter1/1
  [gate_cmd_Q1] -> Simulink-PS Converter/1
  gate_cmds/1 -> Bus Selector/1
  Bus Selector/4 -> [gate_cmd_Q4]  "<gate_cmd_Q4>"
  Bus Selector/3 -> [gate_cmd_Q3]  "<gate_cmd_Q3>"
  Bus Selector/2 -> [gate_cmd_Q2]  "<gate_cmd_Q2>"
  Bus Selector/1 -> [gate_cmd_Q1]  "<gate_cmd_Q1>"
  connections:
  PS-Simulink Converter1/LConn1 -- Voltage Sensor1/RConn1
  Voltage Sensor/RConn1 -- PS-Simulink Converter/LConn1
  igbt_simple_3/RConn1 -- igbt_simple_4/LConn2 -- u2/RConn1 -- Voltage Sensor1/LConn1
  igbt_simple_2/RConn1 -- udc(-)/RConn1 -- igbt_simple_4/RConn1 -- Voltage Sensor1/RConn2 -- Voltage Sensor/RConn2
  igbt_simple_4/LConn1 -- Simulink-PS Converter3/RConn1
  igbt_simple_3/LConn1 -- Simulink-PS Converter2/RConn1
  igbt_simple_2/LConn1 -- Simulink-PS Converter1/RConn1
  igbt_simple_1/LConn1 -- Simulink-PS Converter/RConn1
  udc(+)/RConn1 -- igbt_simple_3/LConn2 -- igbt_simple_1/LConn2
  igbt_simple_1/RConn1 -- igbt_simple_2/LConn2 -- u1/RConn1 -- Voltage Sensor/LConn1

== system single_phase_afe/single_phase_inverter/single phase inverter control/single_phase_inverter_ctrl/dclink_power_decoupling/dclink_decoupling_ctrl ==
  i_dc_buffer_ref : Inport
  udc_dclink_pu : Inport  Port=2
  u_ctrl_out : Inport  Port=3
  Step : Step  Time=param.afe.ctrl.apd.t_enable
  Sum : Sum  Inputs=++|
  alphabeta2dq : Subsystem
  dclink compensation : Scope  NumInputPorts=4
      settings: ActiveDisplayString=3  ActiveDisplayYMinimum=-0.01260398305630173  ActiveDisplayYMaximum=0.11343584750671559  DataLoggingVariableName=ScopeData11
  dclink compensation performance : Scope  NumInputPorts=4
      settings: ActiveDisplayString=3  ActiveDisplayYMinimum=0.50768324908088236  ActiveDisplayYMaximum=1.465576171875  DataLoggingVariableName=ScopeData10
  dq2alphabeta : Subsystem
  dq_vector_pi : Subsystem
      settings: PortSchema="{\"entries\":[{\"content\":{\"sides\":[{\"content\":{\"connectorIds\":[\"In1\",\"In2\"]},\"type\":\"ConnectorPlacement.EquallySpacedRectSide\",\"uuid\":\"dbe4adab-ec2b-4098-a562-e8a7ad70f500\"},{\"content\":{\"connectorIds\":[\"Out1\",\"Out2\"],\"side\":\"RIGHT\"},\"type\":\"ConnectorPlacement.EquallySpacedRectSide\",\"uuid\":\"44034bca-e9c6-4577-a5c6-55d2d85fca45\"},{\"content\":{\"connectorIds\":[\"In3\"],\"side\":\"TOP\"},\"type\":\"ConnectorPlacement.EquallySpacedRectSide\",\"uuid\":\"fe3852dc-ea1e-418a-a8f2-b25375d07ced\"}]},\"type\":\"ConnectorPlacement.EquallySpacedConnector\",\"uuid\":\"21ba8d47-2c84-40ed-8aa8-282f75468d0b\"}],\"packageUris\":[\"http://schema.mathworks.com/mf0/Connector/R2020b\"],\"version\":\"1.0\"}"
  dx_dt : Subsystem
  phase_shift_method_ccaller : Subsystem
  udc_buffer dclink voltage : Scope  NumInputPorts=3
      settings: ActiveDisplayYMinimum=-0.16107177734374997  ActiveDisplayYMaximum=1.44964599609375  DataLoggingVariableName=ScopeData9
  i_buffer_ref : Outport
  tag scope: dclink_buffer_ac_voltage_ctrl_out=scoped, dclink_buffer_dc_voltage_ctrl_out=scoped, dclink_buffer_voltage_ctrl_out=scoped
  wires:
  phase_shift_method_ccaller/1(x_out) -> alphabeta2dq/1(alpha)
  alphabeta2dq/1("dclink_voltage_ripple_d ") -> dclink compensation/1, dq_vector_pi/1(d)  "dclink_voltage_ripple_d"
  alphabeta2dq/2("dclink_voltage_ripple_q ") -> dclink compensation/2, dq_vector_pi/2(q)  "dclink_voltage_ripple_q"
  [udc_buffer] -> udc_buffer dclink voltage/1  "udc_buffer_pu"
  i_dc_buffer_ref/1 -> [dclink_buffer_dc_voltage_ctrl_out], Sum/2
  dx_dt/1(x_hat_ac) -> phase_shift_method_ccaller/1(x_in), dclink compensation performance/2  "udc_hat_pu"
  [phase] -> udc_buffer dclink voltage/3  "phase_ripple"
  dq_vector_pi/1(ud_ctrl_out) -> dclink compensation/3, dq2alphabeta/1(d)  "dclink_voltage_ripple_cmp_ctrl_out_d"
  dq_vector_pi/2(uq_ctrl_out) -> dclink compensation/4, dq2alphabeta/2(q)  "dclink_voltage_ripple_cmp_ctrl_out_q"
  Sum/1 -> [dclink_buffer_voltage_ctrl_out], i_buffer_ref/1, dclink compensation performance/1  "i_buffer_ref"
  phase_shift_method_ccaller/2(y_out) -> alphabeta2dq/2(beta)
  dq2alphabeta/1(i_buffer_ref) -> [dclink_buffer_ac_voltage_ctrl_out], Sum/1  "i_ac_buffer_ref"
  udc_dclink_pu/1 -> udc_buffer dclink voltage/2, dx_dt/1(x), dclink compensation performance/3
  u_ctrl_out/1 -> dclink compensation performance/4  "u_ctrl_out"
  Step/1 -> dq_vector_pi/3(enable)

== system single_phase_afe/single_phase_inverter/single phase inverter control/single_phase_inverter_ctrl/dclink_power_decoupling/idc_buffer_ctrl ==
  i_buffer_ref : Inport
  Bus Creator : BusCreator  Inputs=3
  Gain1 : Gain  Gain=-1
  Gain2 : Gain  Gain=-1
  i_buffer_tracking : Scope
      settings: ActiveDisplayYMinimum=-2.52935791015625  ActiveDisplayYMaximum=1.39215087890625  DataLoggingVariableName=ScopeData17
  pi_ctrl : pi_ctrl/pi_ctrl  kp=param.afe.ctrl.buffer.kp_i  ki=param.afe.ctrl.buffer.ki_i  ts=param.glb_time.ts_afe  lim_up=param.afe.ctrl.buffer.lim_i  lim_down=-param.afe.ctrl.buffer.lim_i
  u_ctrl_out : Outport
  tag scope: dclink_buffer_current_ctrl_out=scoped
  wires:
  [dclink_voltage_pu] -> pi_ctrl/3  "dclink_voltage_pu"
  [i_buffer] -> Gain2/1  "i_buffer"
  i_buffer_ref/1 -> Gain1/1
  Bus Creator/1 -> i_buffer_tracking/1
  pi_ctrl/1 -> [dclink_buffer_current_ctrl_out], u_ctrl_out/1, Bus Creator/3  "u_ctrl_out"
  Gain1/1 -> pi_ctrl/1, Bus Creator/1  "i_buffer_ref"
  Gain2/1 -> pi_ctrl/2, Bus Creator/2  "i_buffer"

== system single_phase_afe/single_phase_inverter/single phase inverter control/single_phase_inverter_ctrl/dclink_power_decoupling/udc_buffer_ctrl ==
  udc_buffer_pu : Inport
  Constant : Constant  Value=0
  discrete-time-low-pass-filter1 : discrete_time_low_pass_filter/discrete-time-low-pass-filter  tau=param.afe.ctrl.buffer.tau_ref  ts=param.glb_time.ts_afe
  pi_ctrl : pi_ctrl/pi_ctrl  kp=param.afe.ctrl.buffer.kp_u  ki=param.afe.ctrl.buffer.ki_u  ts=param.glb_time.ts_afe  lim_up=param.afe.ctrl.buffer.lim_u  lim_down=-param.afe.ctrl.buffer.lim_u
  udc_buffer_norm_ref : Step  Time=param.afe.ctrl.buffer.t_ref  FinalValue=param.afe.ctrl.buffer.udc_pu_ref
  udc_buffer_tracking : Scope  NumInputPorts=3
      settings: ActiveDisplayYMinimum=-1.56976318359375  ActiveDisplayYMaximum=4.12786865234375  DataLoggingVariableName=ScopeData8
  i_dc_buffer_ref : Outport
  wires:
  udc_buffer_norm_ref/1 -> discrete-time-low-pass-filter1/1
  discrete-time-low-pass-filter1/1 -> pi_ctrl/1, udc_buffer_tracking/1  "udc_pu_ref"
  udc_buffer_pu/1 -> pi_ctrl/2, udc_buffer_tracking/2  "udc_pu"
  Constant/1 -> pi_ctrl/3
  pi_ctrl/1 -> i_dc_buffer_ref/1, udc_buffer_tracking/3  "i_dc_buffer_ref"

== system single_phase_afe/single_phase_inverter/single phase inverter control/single_phase_inverter_ctrl/phase PLL/FHT-PLL ==
  ug_abc_pu : Inport
  pll_stageA : Subsystem
  pll_stageB : Subsystem
  phase_grid_fht_pll : Outport
  omega_grid_fht_pll : Outport  Port=2
  wires:
  ug_abc_pu/1 -> pll_stageA/2(ug_abc_pu)
  pll_stageB/2(omega_grid_ddsrf_pll) -> omega_grid_fht_pll/1
  pll_stageA/1(u_grid_xi) -> pll_stageB/1(u_grid_pos_xi)  "u_grid_pos_xi"
  pll_stageA/2(u_grid_eta) -> pll_stageB/2(u_grid_pos_eta)  "u_grid_pos_eta"
  pll_stageB/1(gamma_grid_ddsrf_pll) -> phase_grid_fht_pll/1, pll_stageA/1(gamma_grid)

== system single_phase_afe/single_phase_inverter/single phase inverter control/single_phase_inverter_ctrl/single_phase_current_control/current_reference_generation ==
  i_xi_pu_ref : Inport
  phase : Inport  Port=2
  Bus Creator : BusCreator  Inputs=2
  Product : Product
  Product1 : Product
  Sin : Trigonometry  Operator=cos
  Sin1 : Trigonometry
  is_ref : Outport
  id_ref : Outport  Port=2
  wires:
  Sin/1 -> Product/2
  phase/1 -> Sin1/1, Sin/1
  i_xi_pu_ref/1 -> id_ref/1, Product1/1, Product/1
  Sin1/1 -> Product1/2
  Product/1 -> Bus Creator/1  "is_ref_alpha"
  Product1/1 -> Bus Creator/2  "is_ref_beta"
  Bus Creator/1 -> is_ref/1
